simulink model "Matlab_model"  (R2025b)
settings: Solver=VariableStepAuto  StartTime=0.0  StopTime=10.0  RelTol=1e-3
values from neighbouring files (symbols this model uses):
  g = 9.80665    [init_pendulum.m]
  pin1_angle_rad = deg2rad(pin1_angle)    [init_pendulum.m]
  pin1_damping = 0.025    [init_pendulum.m]
  pin2_angle_rad = deg2rad(pin2_angle)    [init_pendulum.m]
  pin2_damping = 0.01    [init_pendulum.m]
  rod1_Innertia = 0.25 * rod1_mass * (rod1_radius^2) + (1/12) * rod1_mass * (rod1_length^2)    (= 1.78039946165)    [init_pendulum.m]
  rod1_length = 1    [init_pendulum.m]
  rod1_mass = density1*(pi*rod1_radius^2*rod1_length)    (= 21.2057504117)    [init_pendulum.m]
  rod2_Innertia = 0.25 * rod2_mass * (rod2_radius^2) + (1/12) * rod2_mass * (rod2_length^2)    (= 2.15444533697)    [init_pendulum.m]
  rod2_length = 0.75    [init_pendulum.m]
  rod2_mass = density2*(pi*rod2_radius^2*rod2_length)    (= 45.3567439362)    [init_pendulum.m]
settings Model: Creator=Hp  LastModifiedBy=Hp

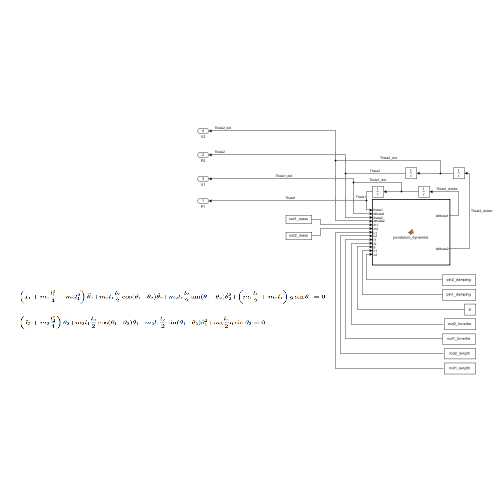
[thumbnail: Simulink's stored preview of the top-level diagram]
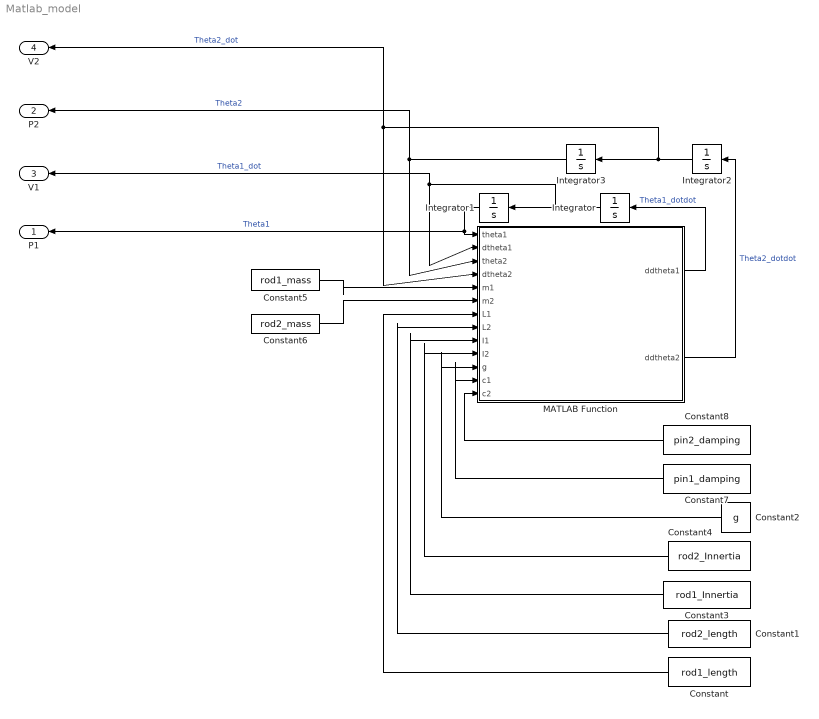
== system Matlab_model ==
  Constant : Constant  Value=rod1_length
  Constant1 : Constant  Value=rod2_length
  Constant2 : Constant  Value=g
  Constant3 : Constant  Value=rod1_Innertia
  Constant4 : Constant  Value=rod2_Innertia
  Constant5 : Constant  Value=rod1_mass
  Constant6 : Constant  Value=rod2_mass
  Constant7 : Constant  Value=pin1_damping
  Constant8 : Constant  Value=pin2_damping
  Integrator : Integrator
  Integrator1 : Integrator  InitialCondition=pin1_angle_rad
  Integrator2 : Integrator
  Integrator3 : Integrator  InitialCondition=pin1_angle_rad + pin2_angle_rad
  MATLAB Function : MATLAB Function  TreatAsAtomicUnit=on
  P1 : Outport  VectorParamsAs1DForOutWhenUnconnected=off
  P2 : Outport  Port=2  VectorParamsAs1DForOutWhenUnconnected=off
  V1 : Outport  Port=3  VectorParamsAs1DForOutWhenUnconnected=off
  V2 : Outport  Port=4  VectorParamsAs1DForOutWhenUnconnected=off
  wires:
  MATLAB Function/2(ddtheta2) -> Integrator2/1  "Theta2_dotdot"
  Integrator/1 -> Integrator1/1, V1/1, MATLAB Function/2(dtheta1)  "Theta1_dot"
  Constant7/1 -> MATLAB Function/12(c1)
  Constant5/1 -> MATLAB Function/5(m1)
  Constant1/1 -> MATLAB Function/8(L2)
  Constant8/1 -> MATLAB Function/13(c2)
  Constant6/1 -> MATLAB Function/6(m2)
  MATLAB Function/1(ddtheta1) -> Integrator/1  "Theta1_dotdot"
  Constant2/1 -> MATLAB Function/11(g)
  Integrator1/1 -> P1/1, MATLAB Function/1(theta1)  "Theta1"
  Integrator3/1 -> P2/1, MATLAB Function/3(theta2)  "Theta2"
  Integrator2/1 -> V2/1, MATLAB Function/4(dtheta2), Integrator3/1  "Theta2_dot"
  Constant4/1 -> MATLAB Function/10(I2)
  Constant/1 -> MATLAB Function/7(L1)
  Constant3/1 -> MATLAB Function/9(I1)

== matlab function Matlab_model/MATLAB Function ==
  data: theta1 input; ddtheta1 output; dtheta1 input; theta2 input; dtheta2 input; m1 input; m2 input; L1 input; L2 input; I1 input; I2 input; g input; ddtheta2 output; c1 input; c2 input
function [ddtheta1, ddtheta2] = pendulum_dynamics(theta1, dtheta1, theta2, dtheta2, m1, m2, L1, L2, I1, I2, g, c1, c2)

    % Mass/Inertia Matrix Elements
    A1 = I1 + m1*(L1^2)/4 + m2*(L1^2);
    A2 = I2 + m2*(L2^2)/4;
    B  = m2 * L1 * (L2/2) * cos(theta1 - theta2);

    % Centripetal & Gravity Terms (using cos() to align with Simscape's Horizontal 0-degree frame)
    C1 = m2 * L1 * (L2/2) * sin(theta1 - theta2) * (dtheta2^2) + (m1*(L1/2) + m2*L1) * g * cos(theta1);
    C2 = -m2 * L1 * (L2/2) * sin(theta1 - theta2) * (dtheta1^2) - m2 * (L2/2) * g * cos(theta2);

    % Damping Torque Terms (Accounting for relative velocity across Joint 2)
    rel_dtheta2 = dtheta2 - dtheta1;
    D1 = c1 * dtheta1 - c2 * rel_dtheta2;
    D2 = c2 * rel_dtheta2;

    % Solve Linear Matrix System: M * [ddtheta1; ddtheta2] = [-C1 - D1; -C2 - D2]
    M = [A1, B; B, A2];
    F = [-(C1 + D1); -(C2 + D2)];

    accel = M \ F;
    ddtheta1 = accel(1);
    ddtheta2 = accel(2);
end
